simulink model "NonlinearThermalFluidMixingTankwithHeater"  (R2026a)
settings: Solver=VariableStepAuto  StopTime=600  MaxStep=0.5
undefined symbols (not defined in the file): A, Cp, p
settings Model: Creator=Wan Farish  LastModifiedBy=Wan Farish

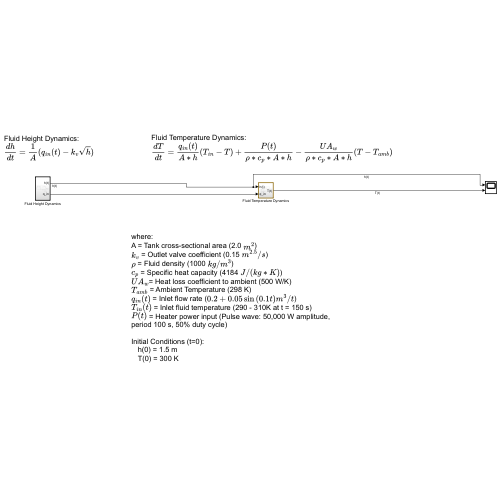
[thumbnail: Simulink's stored preview of the top-level diagram]
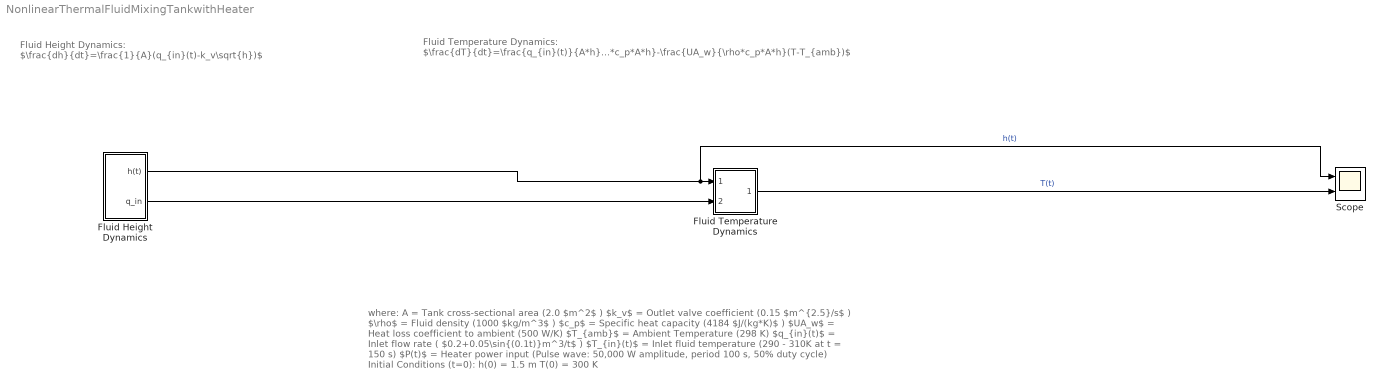
== system NonlinearThermalFluidMixingTankwithHeater ==
  note: where:
      | A = Tank cross-sectional area (2.0 $m^2$ )
      | $k_v$ = Outlet valve coefficient (0.15 $m^{2.5}/s$ )
      | $\rho$ = Fluid density (1000 $kg/m^3$ )
      | $c_p$ = Specific heat capacity (4184 $J/(kg*K)$ )
      | $UA_w$ = Heat loss coefficient to ambient (500 W/K)
      | $T_{amb}$ = Ambient Temperature (298 K)
      | $q_{in}(t)$ = Inlet flow rate ( $0.2+0.05\sin{(0.1t)}m^3/t$ )
      | $T_{in}(t)$ = Inlet fluid temperature (290 - 310K at t = 150 s)
      | $P(t)$ = Heater power input (Pulse wave: 50,000 W amplitude, period 100 s, 50% duty cycle)
      |
      | Initial Conditions (t=0):
      | h(0) = 1.5 m
      | T(0) = 300 K
  note: Fluid Temperature Dynamics:
      | $\frac{dT}{dt}=\frac{q_{in}(t)}{A*h}(T_{in}-T)+\frac{P(t)}{\rho*c_p*A*h}-\frac{UA_w}{\rho*c_p*A*h}(T-T_{amb})$
  note: Fluid Height Dynamics:
      | $\frac{dh}{dt}=\frac{1}{A}(q_{in}(t)-k_v\sqrt{h})$
  Fluid Height Dynamics : Subsystem
  Fluid Temperature Dynamics : Subsystem
  Scope : Scope  NumInputPorts=2
      settings: ActiveDisplayYMinimum=1.4346774880012376  ActiveDisplayYMaximum=2.0879026079888621
  wires:
  Fluid Height Dynamics/1(h(t)) -> Scope/1, Fluid Temperature Dynamics/1(h(t))  "h(t)"
  Fluid Height Dynamics/2(q_in) -> Fluid Temperature Dynamics/2(q_in)
  Fluid Temperature Dynamics/1(T(t)) -> Scope/2  "T(t)"

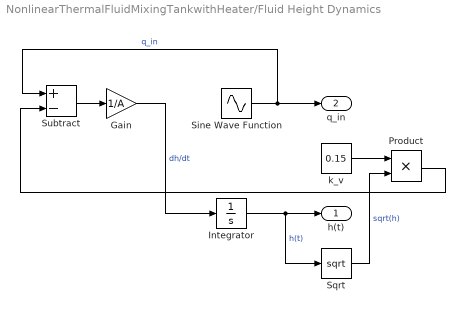
== system NonlinearThermalFluidMixingTankwithHeater/Fluid Height Dynamics ==
  Gain : Gain  Gain=1/A
  Integrator : Integrator  InitialCondition=1.5
  Product : Product
  Sine Wave Function : Sin  Amplitude=0.05  Bias=0.2  Frequency=0.1  SampleTime=0
  Sqrt : Sqrt
  Subtract : Sum  Inputs=+-
  k_v : Constant  Value=0.15
  h(t) : Outport
  q_in : Outport  Port=2
  wires:
  Product/1 -> Subtract/2
  Sqrt/1 -> Product/2  "sqrt(h)"
  k_v/1 -> Product/1
  Gain/1 -> Integrator/1  "dh/dt"
  Subtract/1 -> Gain/1
  Integrator/1 -> h(t)/1, Sqrt/1  "h(t)"
  Sine Wave Function/1 -> Subtract/1, q_in/1  "q_in"

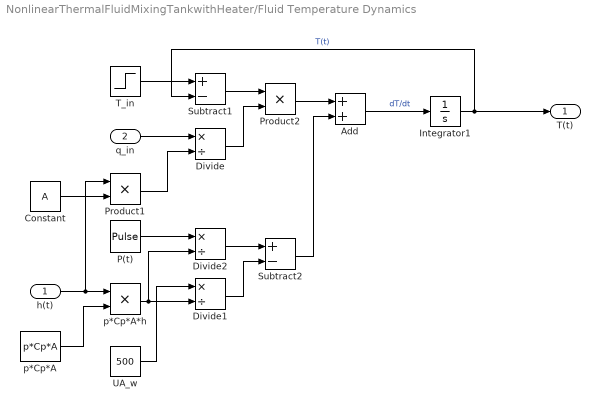
== system NonlinearThermalFluidMixingTankwithHeater/Fluid Temperature Dynamics ==
  h(t) : Inport
  q_in : Inport  Port=2
  Add : Sum
  Constant : Constant  Value=A
  Divide : Product  Inputs=*/
  Divide1 : Product  Inputs=*/
  Divide2 : Product  Inputs=*/
  Integrator1 : Integrator  InitialCondition=300
  P(t) : DiscretePulseGenerator  PulseType=Time based  Amplitude=50000  Period=100  PulseWidth=50
  Product1 : Product
  Product2 : Product
  Subtract1 : Sum  Inputs=+-
  Subtract2 : Sum  Inputs=+-
  T_in : Step  Time=150  InitialValue=290  FinalValue=310  SampleTime=0
  UA_w : Constant  Value=500
  p*Cp*A : Constant  Value=p*Cp*A
  p*Cp*A*h : Product
  T(t) : Outport
  wires:
  Product1/1 -> Divide/2
  Constant/1 -> Product1/2
  T_in/1 -> Subtract1/1
  P(t)/1 -> Divide2/1
  h(t)/1 -> Product1/1, p*Cp*A*h/1
  p*Cp*A/1 -> p*Cp*A*h/2
  q_in/1 -> Divide/1
  p*Cp*A*h/1 -> Divide1/2, Divide2/2
  Subtract1/1 -> Product2/1
  UA_w/1 -> Divide1/1
  Divide/1 -> Product2/2
  Divide2/1 -> Subtract2/1
  Divide1/1 -> Subtract2/2
  Product2/1 -> Add/1
  Subtract2/1 -> Add/2
  Add/1 -> Integrator1/1  "dT/dt"
  Integrator1/1 -> T(t)/1, Subtract1/2  "T(t)"
